simulink model "mars_rover_terrain"  (R2025a)
settings: Solver=daessc  StartTime=0.0  StopTime=130*10  FixedStep=1e-10  MaxStep=1e-1  RelTol=1e-3  AbsTol=1e-3  EnableMultiTasking=on
undefined symbols (not defined in the file): arm_q0, Control, eeConfig, L1, L2, L3, LS1, LS3, R1, R2, R3, Rover, rover_path, RS1, RS3, X, Y, Z
libraries: sm_lib x137, nesl_utility x109, fl_lib x85, sdl_lib x20, ee_lib x10, mars_rover_lib x8, simulink x4, slpidlib x3, batteryecm_lib x2, robotcorelib x1, robotalgslib x1
(part 7 of 10)

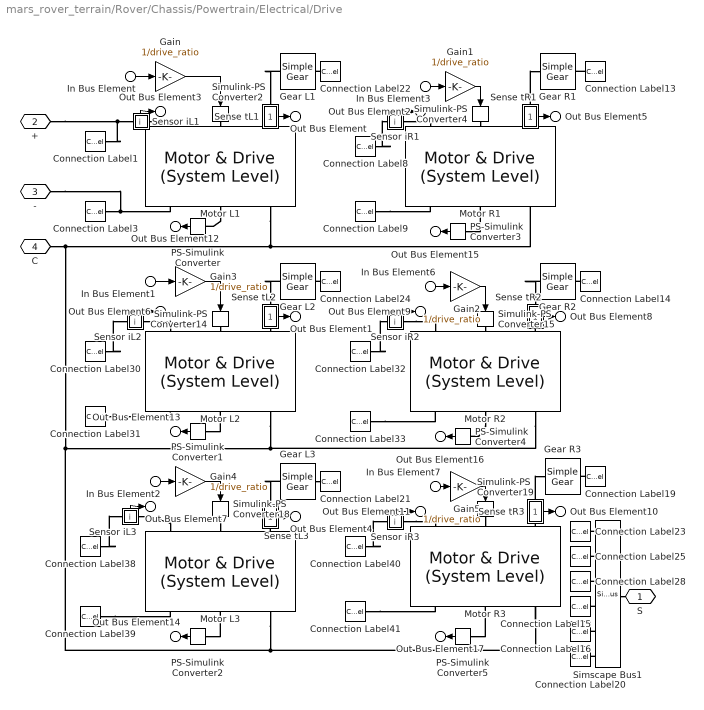
== system mars_rover_terrain/Rover/Chassis/Powertrain/Electrical/Drive ==
  In Bus Element : Inport  PortName=Trq  Element=trq.L1
  In Bus Element1 : Inport  PortName=Trq  Element=trq.L2
  In Bus Element2 : Inport  PortName=Trq  Element=trq.L3
  In Bus Element3 : Inport  PortName=Trq  Element=trq.R1
  In Bus Element6 : Inport  PortName=Trq  Element=trq.R2
  In Bus Element7 : Inport  PortName=Trq  Element=trq.R3
  Connection Label{1,8,30,32,38,40} (6 alike) : ConnectionLabel  Label=p
  Connection Label13 : ConnectionLabel  Label=R1
  Connection Label14 : ConnectionLabel  Label=R2
  Connection Label15 : ConnectionLabel  Label=R1
  Connection Label16 : ConnectionLabel  Label=R2
  Connection Label19 : ConnectionLabel  Label=R3
  Connection Label20 : ConnectionLabel  Label=R3
  Connection Label21 : ConnectionLabel  Label=L3
  Connection Label22 : ConnectionLabel  Label=L1
  Connection Label23 : ConnectionLabel  Label=L1
  Connection Label24 : ConnectionLabel  Label=L2
  Connection Label25 : ConnectionLabel  Label=L2
  Connection Label28 : ConnectionLabel  Label=L3
  Connection Label{3,9,31,33,39,41} (6 alike) : ConnectionLabel  Label=n
  Gain{,1..5} (6 alike) : Gain  Gain=1/drive_ratio
  Gear L2 : sdl_lib/Gears/Simple Gear  ratio=drive_ratio  rotation_direction=sdl.enum.shaftOutputDirection.same  friction_model=sdl.enum.gear_efficiencies_load.off  T_noload=0.1 N*m  T_nom=5 N*m  efficiency_nom=0.8  efficiency=drive_efficiency  temperature_TLU=[280, 300, 320] K  load_TLU=[1, 5, 10] N*m  efficiency_TLU=[.95, .9, .85]  efficiency_TLU2=[.85, .8, .75; .95, .9, .85; .85, .8, .7]  w_thr=0.01 rad/s  pwr_thr=0.001 W  enable_backlash=false  hardstop_model=simscape.enum.hardstop.smooth  backlash_distance=1e-3 mm  r_base=0.1 m  transition=1e-4 mm  backlash_stiffness=1e7 N/m  backlash_damping=1e6 N/(m/s)  coeff_rest=0  v_tol=0.001 m/s  f_tol=0 N  mu_visc=[0, 0] N*m/(rad/s)  thermal_mass=50 J/K  temperature_specify=off  temperature_priority=High  temperature=300 K  temperature_nominal_specify=off  temperature_nominal_value=1  temperature_nominal_unit=K  x_backlash_specify=off  x_backlash_priority=None  x_backlash=0 mm  x_backlash_nominal_specify=off  x_backlash_nominal_value=1  x_backlash_nominal_unit=mm  f_hardstop_specify=off  f_hardstop_priority=None  f_hardstop=0 N  f_hardstop_nominal_specify=off  f_hardstop_nominal_value=1  f_hardstop_nominal_unit=N  v_backlash_specify=off  v_backlash_priority=None  v_backlash=0 m/s  v_backlash_nominal_specify=off  v_backlash_nominal_value=1  v_backlash_nominal_unit=m/s
  Gear L3 : sdl_lib/Gears/Simple Gear  ratio=drive_ratio  rotation_direction=sdl.enum.shaftOutputDirection.same  friction_model=sdl.enum.gear_efficiencies_load.off  T_noload=0.1 N*m  T_nom=5 N*m  efficiency_nom=0.8  efficiency=drive_efficiency  temperature_TLU=[280, 300, 320] K  load_TLU=[1, 5, 10] N*m  efficiency_TLU=[.95, .9, .85]  efficiency_TLU2=[.85, .8, .75; .95, .9, .85; .85, .8, .7]  w_thr=0.01 rad/s  pwr_thr=0.001 W  enable_backlash=false  hardstop_model=simscape.enum.hardstop.smooth  backlash_distance=1e-3 mm  r_base=0.1 m  transition=1e-4 mm  backlash_stiffness=1e7 N/m  backlash_damping=1e6 N/(m/s)  coeff_rest=0  v_tol=0.001 m/s  f_tol=0 N  mu_visc=[0, 0] N*m/(rad/s)  thermal_mass=50 J/K  temperature_specify=off  temperature_priority=High  temperature=300 K  temperature_nominal_specify=off  temperature_nominal_value=1  temperature_nominal_unit=K  x_backlash_specify=off  x_backlash_priority=None  x_backlash=0 mm  x_backlash_nominal_specify=off  x_backlash_nominal_value=1  x_backlash_nominal_unit=mm  f_hardstop_specify=off  f_hardstop_priority=None  f_hardstop=0 N  f_hardstop_nominal_specify=off  f_hardstop_nominal_value=1  f_hardstop_nominal_unit=N  v_backlash_specify=off  v_backlash_priority=None  v_backlash=0 m/s  v_backlash_nominal_specify=off  v_backlash_nominal_value=1  v_backlash_nominal_unit=m/s
  Gear R1 : sdl_lib/Gears/Simple Gear  ratio=drive_ratio  rotation_direction=sdl.enum.shaftOutputDirection.same  friction_model=sdl.enum.gear_efficiencies_load.off  T_noload=0.1 N*m  T_nom=5 N*m  efficiency_nom=0.8  efficiency=drive_efficiency  temperature_TLU=[280, 300, 320] K  load_TLU=[1, 5, 10] N*m  efficiency_TLU=[.95, .9, .85]  efficiency_TLU2=[.85, .8, .75; .95, .9, .85; .85, .8, .7]  w_thr=0.01 rad/s  pwr_thr=0.001 W  enable_backlash=false  hardstop_model=simscape.enum.hardstop.smooth  backlash_distance=1e-3 mm  r_base=0.1 m  transition=1e-4 mm  backlash_stiffness=1e7 N/m  backlash_damping=1e6 N/(m/s)  coeff_rest=0  v_tol=0.001 m/s  f_tol=0 N  mu_visc=[0, 0] N*m/(rad/s)  thermal_mass=50 J/K  temperature_specify=off  temperature_priority=High  temperature=300 K  temperature_nominal_specify=off  temperature_nominal_value=1  temperature_nominal_unit=K  x_backlash_specify=off  x_backlash_priority=None  x_backlash=0 mm  x_backlash_nominal_specify=off  x_backlash_nominal_value=1  x_backlash_nominal_unit=mm  f_hardstop_specify=off  f_hardstop_priority=None  f_hardstop=0 N  f_hardstop_nominal_specify=off  f_hardstop_nominal_value=1  f_hardstop_nominal_unit=N  v_backlash_specify=off  v_backlash_priority=None  v_backlash=0 m/s  v_backlash_nominal_specify=off  v_backlash_nominal_value=1  v_backlash_nominal_unit=m/s
  Gear R2 : sdl_lib/Gears/Simple Gear  ratio=drive_ratio  rotation_direction=sdl.enum.shaftOutputDirection.same  friction_model=sdl.enum.gear_efficiencies_load.off  T_noload=0.1 N*m  T_nom=5 N*m  efficiency_nom=0.8  efficiency=drive_efficiency  temperature_TLU=[280, 300, 320] K  load_TLU=[1, 5, 10] N*m  efficiency_TLU=[.95, .9, .85]  efficiency_TLU2=[.85, .8, .75; .95, .9, .85; .85, .8, .7]  w_thr=0.01 rad/s  pwr_thr=0.001 W  enable_backlash=false  hardstop_model=simscape.enum.hardstop.smooth  backlash_distance=1e-3 mm  r_base=0.1 m  transition=1e-4 mm  backlash_stiffness=1e7 N/m  backlash_damping=1e6 N/(m/s)  coeff_rest=0  v_tol=0.001 m/s  f_tol=0 N  mu_visc=[0, 0] N*m/(rad/s)  thermal_mass=50 J/K  temperature_specify=off  temperature_priority=High  temperature=300 K  temperature_nominal_specify=off  temperature_nominal_value=1  temperature_nominal_unit=K  x_backlash_specify=off  x_backlash_priority=None  x_backlash=0 mm  x_backlash_nominal_specify=off  x_backlash_nominal_value=1  x_backlash_nominal_unit=mm  f_hardstop_specify=off  f_hardstop_priority=None  f_hardstop=0 N  f_hardstop_nominal_specify=off  f_hardstop_nominal_value=1  f_hardstop_nominal_unit=N  v_backlash_specify=off  v_backlash_priority=None  v_backlash=0 m/s  v_backlash_nominal_specify=off  v_backlash_nominal_value=1  v_backlash_nominal_unit=m/s
  Gear R3 : sdl_lib/Gears/Simple Gear  ratio=drive_ratio  rotation_direction=sdl.enum.shaftOutputDirection.same  friction_model=sdl.enum.gear_efficiencies_load.off  T_noload=0.1 N*m  T_nom=5 N*m  efficiency_nom=0.8  efficiency=drive_efficiency  temperature_TLU=[280, 300, 320] K  load_TLU=[1, 5, 10] N*m  efficiency_TLU=[.95, .9, .85]  efficiency_TLU2=[.85, .8, .75; .95, .9, .85; .85, .8, .7]  w_thr=0.01 rad/s  pwr_thr=0.001 W  enable_backlash=false  hardstop_model=simscape.enum.hardstop.smooth  backlash_distance=1e-3 mm  r_base=0.1 m  transition=1e-4 mm  backlash_stiffness=1e7 N/m  backlash_damping=1e6 N/(m/s)  coeff_rest=0  v_tol=0.001 m/s  f_tol=0 N  mu_visc=[0, 0] N*m/(rad/s)  thermal_mass=50 J/K  temperature_specify=off  temperature_priority=High  temperature=300 K  temperature_nominal_specify=off  temperature_nominal_value=1  temperature_nominal_unit=K  x_backlash_specify=off  x_backlash_priority=None  x_backlash=0 mm  x_backlash_nominal_specify=off  x_backlash_nominal_value=1  x_backlash_nominal_unit=mm  f_hardstop_specify=off  f_hardstop_priority=None  f_hardstop=0 N  f_hardstop_nominal_specify=off  f_hardstop_nominal_value=1  f_hardstop_nominal_unit=N  v_backlash_specify=off  v_backlash_priority=None  v_backlash=0 m/s  v_backlash_nominal_specify=off  v_backlash_nominal_value=1  v_backlash_nominal_unit=m/s
  Gear L1 : sdl_lib/Gears/Simple Gear  ratio=drive_ratio  rotation_direction=sdl.enum.shaftOutputDirection.same  friction_model=sdl.enum.gear_efficiencies_load.off  T_noload=0.1 N*m  T_nom=5 N*m  efficiency_nom=0.8  efficiency=drive_efficiency  temperature_TLU=[280, 300, 320] K  load_TLU=[1, 5, 10] N*m  efficiency_TLU=[.95, .9, .85]  efficiency_TLU2=[.85, .8, .75; .95, .9, .85; .85, .8, .7]  w_thr=0.01 rad/s  pwr_thr=0.001 W  enable_backlash=false  hardstop_model=simscape.enum.hardstop.smooth  backlash_distance=1e-3 mm  r_base=0.1 m  transition=1e-4 mm  backlash_stiffness=1e7 N/m  backlash_damping=1e6 N/(m/s)  coeff_rest=0  v_tol=0.001 m/s  f_tol=0 N  mu_visc=[0, 0] N*m/(rad/s)  thermal_mass=50 J/K  temperature_specify=off  temperature_priority=High  temperature=300 K  temperature_nominal_specify=off  temperature_nominal_value=1  temperature_nominal_unit=K  x_backlash_specify=off  x_backlash_priority=None  x_backlash=0 mm  x_backlash_nominal_specify=off  x_backlash_nominal_value=1  x_backlash_nominal_unit=mm  f_hardstop_specify=off  f_hardstop_priority=None  f_hardstop=0 N  f_hardstop_nominal_specify=off  f_hardstop_nominal_value=1  f_hardstop_nominal_unit=N  v_backlash_specify=off  v_backlash_priority=None  v_backlash=0 m/s  v_backlash_nominal_specify=off  v_backlash_nominal_value=1  v_backlash_nominal_unit=m/s
  Motor L1 : ee_lib/Electromechanical/Motor & Drive (System Level)  torque_speed_param=ee.enum.electromech.envelope.torque_power  overtorque_param=ee.enum.electromech.overtorque.no  T_t=[.09, .08, .07, 0] N*m  T_t_intermittent=[.36, .32, .28, 0] N*m  T_t_2D=[.09, .09, .09; .08, .08, .08; .07, .07, .07; 0, 0, 0] N*m  T_t_intermittent_2D=[.36, .36, .36; .32, .32, .32; .28, .28, .28; 0, 0, 0] N*m  w_t=[0, 3750, 7500, 8000] rpm  vdc_t=[6, 12, 24] V  torque_max=trq_max N*m  power_max=power_max W  torque_max_intermittent=0.4 N*m  power_max_intermittent=120 W  time_overtorque=30 s  time_recover=60 s  Tc=trq_tc s  EnableSwitch=simscape.enum.onoff.off  losses_param=1  eff=eff_overall  w_eff=eff_spd rpm  T_eff=eff_trq N*m  Piron=0 % not important in first iteration W  Pbase=0 % not important in first iteration W  w_eff_vec=[-8000, -4000, 0, 4000, 8000] rpm  T_eff_vec=[0, .03, .06, .09] N*m  v_eff_vec=[100, 250, 400] V  losses_mat=[1.49, 1.67, 2.21, 3.1; .42, .69, 1.14, 2.03; .06, .24, .78, 1.68; .42, .69, 1.14, 2.03; 1.49, 1.67, 2.21, 3.1] W  efficiency_mat=[95, 95, 95, 95; 95, 95, 95, 95; 95, 95, 95, 95; 95, 95, 95, 95; 95, 95, 95, 95]  losses_mat_3D=ones(5, 4, 3) W  efficiency_mat_3D=95 * ones(5, 4, 3)  Res=0 % not important in first iteration Ohm  J=0 kg*m^2  lam=rotor_d N*m/(rad/s)  speed0=0 rpm  faulted_specify=off  faulted_priority=None  faulted=0  faulted_nominal_specify=off  faulted_nominal_value=1  faulted_nominal_unit=1  isSwitchedOff_specify=off  isSwitchedOff_priority=None  isSwitchedOff=0  isSwitchedOff_nominal_specify=off  isSwitchedOff_nominal_value=1  isSwitchedOff_nominal_unit=1  torqueLimitContinuous_specify=off  torqueLimitContinuous_priority=None  torqueLimitContinuous=0 N*m  torqueLimitContinuous_nominal_specify=off  torqueLimitContinuous_nominal_value=1  torqueLimitContinuous_nominal_unit=N*m  alpha=3.93e-3 1/K  Tmeas=25 degC  Tmeas2=125 degC  losses_mat_T2=[1.49, 1.74, 2.49, 3.74; .42, .67, 1.42, 2.67; .06, .31, 1.06, 2.31; .42, .67, 1.42, 2.67; 1.49, 1.74, 2.49, 3.74] W  efficiency_mat_T2=[95, 95, 95, 95; 95, 95, 95, 95; 95, 95, 95, 95; 95, 95, 95, 95; 95, 95, 95, 95]  losses_mat_3D_T2=ones(5, 4, 3) W  efficiency_mat_3D_T2=95 * ones(5, 4, 3)  thermal_mass=100 J/K  initial_temperature=25 degC
  Motor L2 : ee_lib/Electromechanical/Motor & Drive (System Level)  torque_speed_param=ee.enum.electromech.envelope.torque_power  overtorque_param=ee.enum.electromech.overtorque.no  T_t=[.09, .08, .07, 0] N*m  T_t_intermittent=[.36, .32, .28, 0] N*m  T_t_2D=[.09, .09, .09; .08, .08, .08; .07, .07, .07; 0, 0, 0] N*m  T_t_intermittent_2D=[.36, .36, .36; .32, .32, .32; .28, .28, .28; 0, 0, 0] N*m  w_t=[0, 3750, 7500, 8000] rpm  vdc_t=[6, 12, 24] V  torque_max=trq_max N*m  power_max=power_max W  torque_max_intermittent=0.4 N*m  power_max_intermittent=120 W  time_overtorque=30 s  time_recover=60 s  Tc=trq_tc s  EnableSwitch=simscape.enum.onoff.off  losses_param=1  eff=eff_overall  w_eff=eff_spd rpm  T_eff=eff_trq N*m  Piron=0 % not important in first iteration W  Pbase=0 % not important in first iteration W  w_eff_vec=[-8000, -4000, 0, 4000, 8000] rpm  T_eff_vec=[0, .03, .06, .09] N*m  v_eff_vec=[100, 250, 400] V  losses_mat=[1.49, 1.67, 2.21, 3.1; .42, .69, 1.14, 2.03; .06, .24, .78, 1.68; .42, .69, 1.14, 2.03; 1.49, 1.67, 2.21, 3.1] W  efficiency_mat=[95, 95, 95, 95; 95, 95, 95, 95; 95, 95, 95, 95; 95, 95, 95, 95; 95, 95, 95, 95]  losses_mat_3D=ones(5, 4, 3) W  efficiency_mat_3D=95 * ones(5, 4, 3)  Res=0 % not important in first iteration Ohm  J=0 kg*m^2  lam=rotor_d N*m/(rad/s)  speed0=0 rpm  faulted_specify=off  faulted_priority=None  faulted=0  faulted_nominal_specify=off  faulted_nominal_value=1  faulted_nominal_unit=1  isSwitchedOff_specify=off  isSwitchedOff_priority=None  isSwitchedOff=0  isSwitchedOff_nominal_specify=off  isSwitchedOff_nominal_value=1  isSwitchedOff_nominal_unit=1  torqueLimitContinuous_specify=off  torqueLimitContinuous_priority=None  torqueLimitContinuous=0 N*m  torqueLimitContinuous_nominal_specify=off  torqueLimitContinuous_nominal_value=1  torqueLimitContinuous_nominal_unit=N*m  alpha=3.93e-3 1/K  Tmeas=25 degC  Tmeas2=125 degC  losses_mat_T2=[1.49, 1.74, 2.49, 3.74; .42, .67, 1.42, 2.67; .06, .31, 1.06, 2.31; .42, .67, 1.42, 2.67; 1.49, 1.74, 2.49, 3.74] W  efficiency_mat_T2=[95, 95, 95, 95; 95, 95, 95, 95; 95, 95, 95, 95; 95, 95, 95, 95; 95, 95, 95, 95]  losses_mat_3D_T2=ones(5, 4, 3) W  efficiency_mat_3D_T2=95 * ones(5, 4, 3)  thermal_mass=100 J/K  initial_temperature=25 degC
  Motor L3 : ee_lib/Electromechanical/Motor & Drive (System Level)  torque_speed_param=ee.enum.electromech.envelope.torque_power  overtorque_param=ee.enum.electromech.overtorque.no  T_t=[.09, .08, .07, 0] N*m  T_t_intermittent=[.36, .32, .28, 0] N*m  T_t_2D=[.09, .09, .09; .08, .08, .08; .07, .07, .07; 0, 0, 0] N*m  T_t_intermittent_2D=[.36, .36, .36; .32, .32, .32; .28, .28, .28; 0, 0, 0] N*m  w_t=[0, 3750, 7500, 8000] rpm  vdc_t=[6, 12, 24] V  torque_max=trq_max N*m  power_max=power_max W  torque_max_intermittent=0.4 N*m  power_max_intermittent=120 W  time_overtorque=30 s  time_recover=60 s  Tc=trq_tc s  EnableSwitch=simscape.enum.onoff.off  losses_param=1  eff=eff_overall  w_eff=eff_spd rpm  T_eff=eff_trq N*m  Piron=0 % not important in first iteration W  Pbase=0 % not important in first iteration W  w_eff_vec=[-8000, -4000, 0, 4000, 8000] rpm  T_eff_vec=[0, .03, .06, .09] N*m  v_eff_vec=[100, 250, 400] V  losses_mat=[1.49, 1.67, 2.21, 3.1; .42, .69, 1.14, 2.03; .06, .24, .78, 1.68; .42, .69, 1.14, 2.03; 1.49, 1.67, 2.21, 3.1] W  efficiency_mat=[95, 95, 95, 95; 95, 95, 95, 95; 95, 95, 95, 95; 95, 95, 95, 95; 95, 95, 95, 95]  losses_mat_3D=ones(5, 4, 3) W  efficiency_mat_3D=95 * ones(5, 4, 3)  Res=0 % not important in first iteration Ohm  J=0 kg*m^2  lam=rotor_d N*m/(rad/s)  speed0=0 rpm  faulted_specify=off  faulted_priority=None  faulted=0  faulted_nominal_specify=off  faulted_nominal_value=1  faulted_nominal_unit=1  isSwitchedOff_specify=off  isSwitchedOff_priority=None  isSwitchedOff=0  isSwitchedOff_nominal_specify=off  isSwitchedOff_nominal_value=1  isSwitchedOff_nominal_unit=1  torqueLimitContinuous_specify=off  torqueLimitContinuous_priority=None  torqueLimitContinuous=0 N*m  torqueLimitContinuous_nominal_specify=off  torqueLimitContinuous_nominal_value=1  torqueLimitContinuous_nominal_unit=N*m  alpha=3.93e-3 1/K  Tmeas=25 degC  Tmeas2=125 degC  losses_mat_T2=[1.49, 1.74, 2.49, 3.74; .42, .67, 1.42, 2.67; .06, .31, 1.06, 2.31; .42, .67, 1.42, 2.67; 1.49, 1.74, 2.49, 3.74] W  efficiency_mat_T2=[95, 95, 95, 95; 95, 95, 95, 95; 95, 95, 95, 95; 95, 95, 95, 95; 95, 95, 95, 95]  losses_mat_3D_T2=ones(5, 4, 3) W  efficiency_mat_3D_T2=95 * ones(5, 4, 3)  thermal_mass=100 J/K  initial_temperature=25 degC
  Motor R1 : ee_lib/Electromechanical/Motor & Drive (System Level)  torque_speed_param=ee.enum.electromech.envelope.torque_power  overtorque_param=ee.enum.electromech.overtorque.no  T_t=[.09, .08, .07, 0] N*m  T_t_intermittent=[.36, .32, .28, 0] N*m  T_t_2D=[.09, .09, .09; .08, .08, .08; .07, .07, .07; 0, 0, 0] N*m  T_t_intermittent_2D=[.36, .36, .36; .32, .32, .32; .28, .28, .28; 0, 0, 0] N*m  w_t=[0, 3750, 7500, 8000] rpm  vdc_t=[6, 12, 24] V  torque_max=trq_max N*m  power_max=power_max W  torque_max_intermittent=0.4 N*m  power_max_intermittent=120 W  time_overtorque=30 s  time_recover=60 s  Tc=trq_tc s  EnableSwitch=simscape.enum.onoff.off  losses_param=1  eff=eff_overall  w_eff=eff_spd rpm  T_eff=eff_trq N*m  Piron=0 % not important in first iteration W  Pbase=0 % not important in first iteration W  w_eff_vec=[-8000, -4000, 0, 4000, 8000] rpm  T_eff_vec=[0, .03, .06, .09] N*m  v_eff_vec=[100, 250, 400] V  losses_mat=[1.49, 1.67, 2.21, 3.1; .42, .69, 1.14, 2.03; .06, .24, .78, 1.68; .42, .69, 1.14, 2.03; 1.49, 1.67, 2.21, 3.1] W  efficiency_mat=[95, 95, 95, 95; 95, 95, 95, 95; 95, 95, 95, 95; 95, 95, 95, 95; 95, 95, 95, 95]  losses_mat_3D=ones(5, 4, 3) W  efficiency_mat_3D=95 * ones(5, 4, 3)  Res=0 % not important in first iteration Ohm  J=0 kg*m^2  lam=rotor_d N*m/(rad/s)  speed0=0 rpm  faulted_specify=off  faulted_priority=None  faulted=0  faulted_nominal_specify=off  faulted_nominal_value=1  faulted_nominal_unit=1  isSwitchedOff_specify=off  isSwitchedOff_priority=None  isSwitchedOff=0  isSwitchedOff_nominal_specify=off  isSwitchedOff_nominal_value=1  isSwitchedOff_nominal_unit=1  torqueLimitContinuous_specify=off  torqueLimitContinuous_priority=None  torqueLimitContinuous=0 N*m  torqueLimitContinuous_nominal_specify=off  torqueLimitContinuous_nominal_value=1  torqueLimitContinuous_nominal_unit=N*m  alpha=3.93e-3 1/K  Tmeas=25 degC  Tmeas2=125 degC  losses_mat_T2=[1.49, 1.74, 2.49, 3.74; .42, .67, 1.42, 2.67; .06, .31, 1.06, 2.31; .42, .67, 1.42, 2.67; 1.49, 1.74, 2.49, 3.74] W  efficiency_mat_T2=[95, 95, 95, 95; 95, 95, 95, 95; 95, 95, 95, 95; 95, 95, 95, 95; 95, 95, 95, 95]  losses_mat_3D_T2=ones(5, 4, 3) W  efficiency_mat_3D_T2=95 * ones(5, 4, 3)  thermal_mass=100 J/K  initial_temperature=25 degC
  Motor R2 : ee_lib/Electromechanical/Motor & Drive (System Level)  torque_speed_param=ee.enum.electromech.envelope.torque_power  overtorque_param=ee.enum.electromech.overtorque.no  T_t=[.09, .08, .07, 0] N*m  T_t_intermittent=[.36, .32, .28, 0] N*m  T_t_2D=[.09, .09, .09; .08, .08, .08; .07, .07, .07; 0, 0, 0] N*m  T_t_intermittent_2D=[.36, .36, .36; .32, .32, .32; .28, .28, .28; 0, 0, 0] N*m  w_t=[0, 3750, 7500, 8000] rpm  vdc_t=[6, 12, 24] V  torque_max=trq_max N*m  power_max=power_max W  torque_max_intermittent=0.4 N*m  power_max_intermittent=120 W  time_overtorque=30 s  time_recover=60 s  Tc=trq_tc s  EnableSwitch=simscape.enum.onoff.off  losses_param=1  eff=eff_overall  w_eff=eff_spd rpm  T_eff=eff_trq N*m  Piron=0 % not important in first iteration W  Pbase=0 % not important in first iteration W  w_eff_vec=[-8000, -4000, 0, 4000, 8000] rpm  T_eff_vec=[0, .03, .06, .09] N*m  v_eff_vec=[100, 250, 400] V  losses_mat=[1.49, 1.67, 2.21, 3.1; .42, .69, 1.14, 2.03; .06, .24, .78, 1.68; .42, .69, 1.14, 2.03; 1.49, 1.67, 2.21, 3.1] W  efficiency_mat=[95, 95, 95, 95; 95, 95, 95, 95; 95, 95, 95, 95; 95, 95, 95, 95; 95, 95, 95, 95]  losses_mat_3D=ones(5, 4, 3) W  efficiency_mat_3D=95 * ones(5, 4, 3)  Res=0 % not important in first iteration Ohm  J=0 kg*m^2  lam=rotor_d N*m/(rad/s)  speed0=0 rpm  faulted_specify=off  faulted_priority=None  faulted=0  faulted_nominal_specify=off  faulted_nominal_value=1  faulted_nominal_unit=1  isSwitchedOff_specify=off  isSwitchedOff_priority=None  isSwitchedOff=0  isSwitchedOff_nominal_specify=off  isSwitchedOff_nominal_value=1  isSwitchedOff_nominal_unit=1  torqueLimitContinuous_specify=off  torqueLimitContinuous_priority=None  torqueLimitContinuous=0 N*m  torqueLimitContinuous_nominal_specify=off  torqueLimitContinuous_nominal_value=1  torqueLimitContinuous_nominal_unit=N*m  alpha=3.93e-3 1/K  Tmeas=25 degC  Tmeas2=125 degC  losses_mat_T2=[1.49, 1.74, 2.49, 3.74; .42, .67, 1.42, 2.67; .06, .31, 1.06, 2.31; .42, .67, 1.42, 2.67; 1.49, 1.74, 2.49, 3.74] W  efficiency_mat_T2=[95, 95, 95, 95; 95, 95, 95, 95; 95, 95, 95, 95; 95, 95, 95, 95; 95, 95, 95, 95]  losses_mat_3D_T2=ones(5, 4, 3) W  efficiency_mat_3D_T2=95 * ones(5, 4, 3)  thermal_mass=100 J/K  initial_temperature=25 degC
  Motor R3 : ee_lib/Electromechanical/Motor & Drive (System Level)  torque_speed_param=ee.enum.electromech.envelope.torque_power  overtorque_param=ee.enum.electromech.overtorque.no  T_t=[.09, .08, .07, 0] N*m  T_t_intermittent=[.36, .32, .28, 0] N*m  T_t_2D=[.09, .09, .09; .08, .08, .08; .07, .07, .07; 0, 0, 0] N*m  T_t_intermittent_2D=[.36, .36, .36; .32, .32, .32; .28, .28, .28; 0, 0, 0] N*m  w_t=[0, 3750, 7500, 8000] rpm  vdc_t=[6, 12, 24] V  torque_max=trq_max N*m  power_max=power_max W  torque_max_intermittent=0.4 N*m  power_max_intermittent=120 W  time_overtorque=30 s  time_recover=60 s  Tc=trq_tc s  EnableSwitch=simscape.enum.onoff.off  losses_param=1  eff=eff_overall  w_eff=eff_spd rpm  T_eff=eff_trq N*m  Piron=0 % not important in first iteration W  Pbase=0 % not important in first iteration W  w_eff_vec=[-8000, -4000, 0, 4000, 8000] rpm  T_eff_vec=[0, .03, .06, .09] N*m  v_eff_vec=[100, 250, 400] V  losses_mat=[1.49, 1.67, 2.21, 3.1; .42, .69, 1.14, 2.03; .06, .24, .78, 1.68; .42, .69, 1.14, 2.03; 1.49, 1.67, 2.21, 3.1] W  efficiency_mat=[95, 95, 95, 95; 95, 95, 95, 95; 95, 95, 95, 95; 95, 95, 95, 95; 95, 95, 95, 95]  losses_mat_3D=ones(5, 4, 3) W  efficiency_mat_3D=95 * ones(5, 4, 3)  Res=0 % not important in first iteration Ohm  J=0 kg*m^2  lam=rotor_d N*m/(rad/s)  speed0=0 rpm  faulted_specify=off  faulted_priority=None  faulted=0  faulted_nominal_specify=off  faulted_nominal_value=1  faulted_nominal_unit=1  isSwitchedOff_specify=off  isSwitchedOff_priority=None  isSwitchedOff=0  isSwitchedOff_nominal_specify=off  isSwitchedOff_nominal_value=1  isSwitchedOff_nominal_unit=1  torqueLimitContinuous_specify=off  torqueLimitContinuous_priority=None  torqueLimitContinuous=0 N*m  torqueLimitContinuous_nominal_specify=off  torqueLimitContinuous_nominal_value=1  torqueLimitContinuous_nominal_unit=N*m  alpha=3.93e-3 1/K  Tmeas=25 degC  Tmeas2=125 degC  losses_mat_T2=[1.49, 1.74, 2.49, 3.74; .42, .67, 1.42, 2.67; .06, .31, 1.06, 2.31; .42, .67, 1.42, 2.67; 1.49, 1.74, 2.49, 3.74] W  efficiency_mat_T2=[95, 95, 95, 95; 95, 95, 95, 95; 95, 95, 95, 95; 95, 95, 95, 95; 95, 95, 95, 95]  losses_mat_3D_T2=ones(5, 4, 3) W  efficiency_mat_3D_T2=95 * ones(5, 4, 3)  thermal_mass=100 J/K  initial_temperature=25 degC
  PS-Simulink Converter{,1..5} (6 alike) : nesl_utility/PS-Simulink Converter  PhysicalDomain=network_engine_domain  SubClassName=ps_output  LeftPortType=input  RightPortType=output  PseudoPeriodic=off  Frequencies=[]  VectorFormat=1-D array  Unit=inherit  AffineConversion=off
  Sense tL1 : Subsystem
      settings: PortSchema="{\"entries\":[{\"content\":{\"sides\":[{\"content\":{\"connectorIds\":[\"LConn1\"]},\"type\":\"ConnectorPlacement.EquallySpacedRectSide\",\"uuid\":\"592cc1a1-656f-47ce-ad3a-4b4dc1070b5c\"},{\"content\":{\"connectorIds\":[\"RConn1\"],\"side\":\"RIGHT\"},\"type\":\"ConnectorPlacement.EquallySpacedRectSide\",\"uuid\":\"9bca39c3-eeb4-4456-9b97-61ec2f027d42\"},{\"content\":{\"connectorIds\":[\"Out1\"],\"side\":\"TOP\"},\"type\":\"ConnectorPlacement.EquallySpacedRectSide\",\"uuid\":\"1e04bf27-fb0c-4be4-96d5-7a7c6152a7df\"}]},\"type\":\"ConnectorPlacement.EquallySpacedConnector\",\"uuid\":\"70eba8cc-e966-48e4-a1ce-5ccb9693dc60\"}],\"packageUris\":[\"http://schema.mathworks.com/mf0/Connector/R2020b\"],\"version\":\"1.0\"}"
      mask Display: disp('t')
  Sense tL2 : Subsystem
      settings: PortSchema="{\"entries\":[{\"content\":{\"sides\":[{\"content\":{\"connectorIds\":[\"LConn1\"]},\"type\":\"ConnectorPlacement.EquallySpacedRectSide\",\"uuid\":\"592cc1a1-656f-47ce-ad3a-4b4dc1070b5c\"},{\"content\":{\"connectorIds\":[\"RConn1\"],\"side\":\"RIGHT\"},\"type\":\"ConnectorPlacement.EquallySpacedRectSide\",\"uuid\":\"9bca39c3-eeb4-4456-9b97-61ec2f027d42\"},{\"content\":{\"connectorIds\":[\"Out1\"],\"side\":\"TOP\"},\"type\":\"ConnectorPlacement.EquallySpacedRectSide\",\"uuid\":\"1e04bf27-fb0c-4be4-96d5-7a7c6152a7df\"}]},\"type\":\"ConnectorPlacement.EquallySpacedConnector\",\"uuid\":\"70eba8cc-e966-48e4-a1ce-5ccb9693dc60\"}],\"packageUris\":[\"http://schema.mathworks.com/mf0/Connector/R2020b\"],\"version\":\"1.0\"}"
      mask Display: disp('t')
  Sense tL3 : Subsystem
      settings: PortSchema="{\"entries\":[{\"content\":{\"sides\":[{\"content\":{\"connectorIds\":[\"LConn1\"]},\"type\":\"ConnectorPlacement.EquallySpacedRectSide\",\"uuid\":\"592cc1a1-656f-47ce-ad3a-4b4dc1070b5c\"},{\"content\":{\"connectorIds\":[\"RConn1\"],\"side\":\"RIGHT\"},\"type\":\"ConnectorPlacement.EquallySpacedRectSide\",\"uuid\":\"9bca39c3-eeb4-4456-9b97-61ec2f027d42\"},{\"content\":{\"connectorIds\":[\"Out1\"],\"side\":\"TOP\"},\"type\":\"ConnectorPlacement.EquallySpacedRectSide\",\"uuid\":\"1e04bf27-fb0c-4be4-96d5-7a7c6152a7df\"},{\"content\":{\"connectorIds\":[],\"side\":\"BOTTOM\"},\"type\":\"ConnectorPlacement.EquallySpacedRectSide\",\"uuid\":\"710085da-f7c8-4ce8-b21c-6bd8281c2790\"}]},\"type\":\"ConnectorPlacement.EquallySpacedConnector\",\"uuid\":\"70eba8cc-e966-48e4-a1ce-5ccb9693dc60\"}],\"packageUris\":[\"http://schema.mathworks.com/mf0/Connector/R2020b\"],\"version\":\"1.0\"}"
      mask Display: disp('t')
  Sense tR1 : Subsystem
      settings: PortSchema="{\"entries\":[{\"content\":{\"sides\":[{\"content\":{\"connectorIds\":[\"LConn1\"]},\"type\":\"ConnectorPlacement.EquallySpacedRectSide\",\"uuid\":\"592cc1a1-656f-47ce-ad3a-4b4dc1070b5c\"},{\"content\":{\"connectorIds\":[\"RConn1\"],\"side\":\"RIGHT\"},\"type\":\"ConnectorPlacement.EquallySpacedRectSide\",\"uuid\":\"9bca39c3-eeb4-4456-9b97-61ec2f027d42\"},{\"content\":{\"connectorIds\":[\"Out1\"],\"side\":\"TOP\"},\"type\":\"ConnectorPlacement.EquallySpacedRectSide\",\"uuid\":\"1e04bf27-fb0c-4be4-96d5-7a7c6152a7df\"}]},\"type\":\"ConnectorPlacement.EquallySpacedConnector\",\"uuid\":\"70eba8cc-e966-48e4-a1ce-5ccb9693dc60\"}],\"packageUris\":[\"http://schema.mathworks.com/mf0/Connector/R2020b\"],\"version\":\"1.0\"}"
      mask Display: disp('t')
  Sense tR2 : Subsystem
      settings: PortSchema="{\"entries\":[{\"content\":{\"sides\":[{\"content\":{\"connectorIds\":[\"LConn1\"]},\"type\":\"ConnectorPlacement.EquallySpacedRectSide\",\"uuid\":\"592cc1a1-656f-47ce-ad3a-4b4dc1070b5c\"},{\"content\":{\"connectorIds\":[\"RConn1\"],\"side\":\"RIGHT\"},\"type\":\"ConnectorPlacement.EquallySpacedRectSide\",\"uuid\":\"9bca39c3-eeb4-4456-9b97-61ec2f027d42\"},{\"content\":{\"connectorIds\":[\"Out1\"],\"side\":\"TOP\"},\"type\":\"ConnectorPlacement.EquallySpacedRectSide\",\"uuid\":\"1e04bf27-fb0c-4be4-96d5-7a7c6152a7df\"}]},\"type\":\"ConnectorPlacement.EquallySpacedConnector\",\"uuid\":\"70eba8cc-e966-48e4-a1ce-5ccb9693dc60\"}],\"packageUris\":[\"http://schema.mathworks.com/mf0/Connector/R2020b\"],\"version\":\"1.0\"}"
      mask Display: disp('t')
  Sense tR3 : Subsystem
      settings: PortSchema="{\"entries\":[{\"content\":{\"sides\":[{\"content\":{\"connectorIds\":[\"LConn1\"]},\"type\":\"ConnectorPlacement.EquallySpacedRectSide\",\"uuid\":\"592cc1a1-656f-47ce-ad3a-4b4dc1070b5c\"},{\"content\":{\"connectorIds\":[\"RConn1\"],\"side\":\"RIGHT\"},\"type\":\"ConnectorPlacement.EquallySpacedRectSide\",\"uuid\":\"9bca39c3-eeb4-4456-9b97-61ec2f027d42\"},{\"content\":{\"connectorIds\":[\"Out1\"],\"side\":\"TOP\"},\"type\":\"ConnectorPlacement.EquallySpacedRectSide\",\"uuid\":\"1e04bf27-fb0c-4be4-96d5-7a7c6152a7df\"}]},\"type\":\"ConnectorPlacement.EquallySpacedConnector\",\"uuid\":\"70eba8cc-e966-48e4-a1ce-5ccb9693dc60\"}],\"packageUris\":[\"http://schema.mathworks.com/mf0/Connector/R2020b\"],\"version\":\"1.0\"}"
      mask Display: disp('t')
  Sensor iL1 : Subsystem
      settings: PortSchema="{\"entries\":[{\"content\":{\"sides\":[{\"content\":{\"connectorIds\":[\"LConn1\"]},\"type\":\"ConnectorPlacement.EquallySpacedRectSide\",\"uuid\":\"592cc1a1-656f-47ce-ad3a-4b4dc1070b5c\"},{\"content\":{\"connectorIds\":[\"RConn1\"],\"side\":\"RIGHT\"},\"type\":\"ConnectorPlacement.EquallySpacedRectSide\",\"uuid\":\"9bca39c3-eeb4-4456-9b97-61ec2f027d42\"},{\"content\":{\"connectorIds\":[\"Out1\"],\"side\":\"TOP\"},\"type\":\"ConnectorPlacement.EquallySpacedRectSide\",\"uuid\":\"1e04bf27-fb0c-4be4-96d5-7a7c6152a7df\"}]},\"type\":\"ConnectorPlacement.EquallySpacedConnector\",\"uuid\":\"70eba8cc-e966-48e4-a1ce-5ccb9693dc60\"}],\"packageUris\":[\"http://schema.mathworks.com/mf0/Connector/R2020b\"],\"version\":\"1.0\"}"
      mask Display: disp('i');
  Sensor iL2 : Subsystem
      settings: PortSchema="{\"entries\":[{\"content\":{\"sides\":[{\"content\":{\"connectorIds\":[\"LConn1\"]},\"type\":\"ConnectorPlacement.EquallySpacedRectSide\",\"uuid\":\"592cc1a1-656f-47ce-ad3a-4b4dc1070b5c\"},{\"content\":{\"connectorIds\":[\"RConn1\"],\"side\":\"RIGHT\"},\"type\":\"ConnectorPlacement.EquallySpacedRectSide\",\"uuid\":\"9bca39c3-eeb4-4456-9b97-61ec2f027d42\"},{\"content\":{\"connectorIds\":[\"Out1\"],\"side\":\"TOP\"},\"type\":\"ConnectorPlacement.EquallySpacedRectSide\",\"uuid\":\"1e04bf27-fb0c-4be4-96d5-7a7c6152a7df\"}]},\"type\":\"ConnectorPlacement.EquallySpacedConnector\",\"uuid\":\"70eba8cc-e966-48e4-a1ce-5ccb9693dc60\"}],\"packageUris\":[\"http://schema.mathworks.com/mf0/Connector/R2020b\"],\"version\":\"1.0\"}"
      mask Display: disp('i');
  Sensor iL3 : Subsystem
      settings: PortSchema="{\"entries\":[{\"content\":{\"sides\":[{\"content\":{\"connectorIds\":[\"LConn1\"]},\"type\":\"ConnectorPlacement.EquallySpacedRectSide\",\"uuid\":\"592cc1a1-656f-47ce-ad3a-4b4dc1070b5c\"},{\"content\":{\"connectorIds\":[\"RConn1\"],\"side\":\"RIGHT\"},\"type\":\"ConnectorPlacement.EquallySpacedRectSide\",\"uuid\":\"9bca39c3-eeb4-4456-9b97-61ec2f027d42\"},{\"content\":{\"connectorIds\":[\"Out1\"],\"side\":\"TOP\"},\"type\":\"ConnectorPlacement.EquallySpacedRectSide\",\"uuid\":\"1e04bf27-fb0c-4be4-96d5-7a7c6152a7df\"}]},\"type\":\"ConnectorPlacement.EquallySpacedConnector\",\"uuid\":\"70eba8cc-e966-48e4-a1ce-5ccb9693dc60\"}],\"packageUris\":[\"http://schema.mathworks.com/mf0/Connector/R2020b\"],\"version\":\"1.0\"}"
      mask Display: disp('i');
  Sensor iR1 : Subsystem
      settings: PortSchema="{\"entries\":[{\"content\":{\"sides\":[{\"content\":{\"connectorIds\":[\"LConn1\"]},\"type\":\"ConnectorPlacement.EquallySpacedRectSide\",\"uuid\":\"592cc1a1-656f-47ce-ad3a-4b4dc1070b5c\"},{\"content\":{\"connectorIds\":[\"RConn1\"],\"side\":\"RIGHT\"},\"type\":\"ConnectorPlacement.EquallySpacedRectSide\",\"uuid\":\"9bca39c3-eeb4-4456-9b97-61ec2f027d42\"},{\"content\":{\"connectorIds\":[\"Out1\"],\"side\":\"TOP\"},\"type\":\"ConnectorPlacement.EquallySpacedRectSide\",\"uuid\":\"1e04bf27-fb0c-4be4-96d5-7a7c6152a7df\"}]},\"type\":\"ConnectorPlacement.EquallySpacedConnector\",\"uuid\":\"70eba8cc-e966-48e4-a1ce-5ccb9693dc60\"}],\"packageUris\":[\"http://schema.mathworks.com/mf0/Connector/R2020b\"],\"version\":\"1.0\"}"
      mask Display: disp('i');
  Sensor iR2 : Subsystem
      settings: PortSchema="{\"entries\":[{\"content\":{\"sides\":[{\"content\":{\"connectorIds\":[\"LConn1\"]},\"type\":\"ConnectorPlacement.EquallySpacedRectSide\",\"uuid\":\"592cc1a1-656f-47ce-ad3a-4b4dc1070b5c\"},{\"content\":{\"connectorIds\":[\"RConn1\"],\"side\":\"RIGHT\"},\"type\":\"ConnectorPlacement.EquallySpacedRectSide\",\"uuid\":\"9bca39c3-eeb4-4456-9b97-61ec2f027d42\"},{\"content\":{\"connectorIds\":[\"Out1\"],\"side\":\"TOP\"},\"type\":\"ConnectorPlacement.EquallySpacedRectSide\",\"uuid\":\"1e04bf27-fb0c-4be4-96d5-7a7c6152a7df\"}]},\"type\":\"ConnectorPlacement.EquallySpacedConnector\",\"uuid\":\"70eba8cc-e966-48e4-a1ce-5ccb9693dc60\"}],\"packageUris\":[\"http://schema.mathworks.com/mf0/Connector/R2020b\"],\"version\":\"1.0\"}"
      mask Display: disp('i');
  Sensor iR3 : Subsystem
      settings: PortSchema="{\"entries\":[{\"content\":{\"sides\":[{\"content\":{\"connectorIds\":[\"LConn1\"]},\"type\":\"ConnectorPlacement.EquallySpacedRectSide\",\"uuid\":\"592cc1a1-656f-47ce-ad3a-4b4dc1070b5c\"},{\"content\":{\"connectorIds\":[\"RConn1\"],\"side\":\"RIGHT\"},\"type\":\"ConnectorPlacement.EquallySpacedRectSide\",\"uuid\":\"9bca39c3-eeb4-4456-9b97-61ec2f027d42\"},{\"content\":{\"connectorIds\":[\"Out1\"],\"side\":\"TOP\"},\"type\":\"ConnectorPlacement.EquallySpacedRectSide\",\"uuid\":\"1e04bf27-fb0c-4be4-96d5-7a7c6152a7df\"}]},\"type\":\"ConnectorPlacement.EquallySpacedConnector\",\"uuid\":\"70eba8cc-e966-48e4-a1ce-5ccb9693dc60\"}],\"packageUris\":[\"http://schema.mathworks.com/mf0/Connector/R2020b\"],\"version\":\"1.0\"}"
      mask Display: disp('i');
  Simscape Bus1 : SimscapeBus  HierarchyStrings=L1;L2;L3;R1;R2;R3
  Simulink-PS Converter{2,4,14..15,18..19} (6 alike) : nesl_utility/Simulink-PS Converter  PhysicalDomain=network_engine_domain  SubClassName=ps_input  LeftPortType=input  RightPortType=output  PseudoPeriodic=off  Frequencies=[]  NoiseDistribution=none  NoiseParameters=[]  Unit=N*m  AffineConversion=off  FilteringAndDerivatives=provide  SimscapeFilterOrder=1  InputFilterTimeConstant=0.001  UdotUserProvided=0
  S : PMIOPort  Side=Right
  + : PMIOPort  Port=2  Side=Left
  - : PMIOPort  Port=3  Side=Left
  C : PMIOPort  Port=4  Side=Right
  Out Bus Element : Outport  PortName=m  Element=trq.L1
  Out Bus Element1 : Outport  PortName=m  Element=trq.L2
  Out Bus Element4 : Outport  PortName=m  Element=trq.L3
  Out Bus Element5 : Outport  PortName=m  Element=trq.R1
  Out Bus Element8 : Outport  PortName=m  Element=trq.R2
  Out Bus Element10 : Outport  PortName=m  Element=trq.R3
  Out Bus Element3 : Outport  PortName=m  Element=i.L1
  Out Bus Element6 : Outport  PortName=m  Element=i.L2
  Out Bus Element7 : Outport  PortName=m  Element=i.L3
  Out Bus Element2 : Outport  PortName=m  Element=i.R1
  Out Bus Element9 : Outport  PortName=m  Element=i.R2
  Out Bus Element11 : Outport  PortName=m  Element=i.R3
  Out Bus Element12 : Outport  PortName=m  Element=w.L1
  Out Bus Element13 : Outport  PortName=m  Element=w.L2
  Out Bus Element14 : Outport  PortName=m  Element=w.L3
  Out Bus Element15 : Outport  PortName=m  Element=w.R1
  Out Bus Element16 : Outport  PortName=m  Element=w.R2
  Out Bus Element17 : Outport  PortName=m  Element=w.R3
  wires:
  Sensor iR2/1(i) -> Out Bus Element9/1
  Sensor iL1/1(i) -> Out Bus Element3/1
  Sensor iL3/1(i) -> Out Bus Element7/1
  Sensor iL2/1(i) -> Out Bus Element6/1
  Sensor iR1/1(i) -> Out Bus Element2/1
  In Bus Element/1 -> Gain/1
  In Bus Element1/1 -> Gain3/1
  In Bus Element2/1 -> Gain4/1
  In Bus Element3/1 -> Gain1/1
  In Bus Element6/1 -> Gain2/1
  In Bus Element7/1 -> Gain5/1
  Sensor iR3/1(i) -> Out Bus Element11/1
  Gain/1 -> Simulink-PS Converter2/1
  Gain1/1 -> Simulink-PS Converter4/1
  Gain2/1 -> Simulink-PS Converter15/1
  Gain3/1 -> Simulink-PS Converter14/1
  Gain4/1 -> Simulink-PS Converter18/1
  Gain5/1 -> Simulink-PS Converter19/1
  Sense tL1/1(T) -> Out Bus Element/1
  Sense tR1/1(T) -> Out Bus Element5/1
  PS-Simulink Converter/1 -> Out Bus Element12/1
  PS-Simulink Converter1/1 -> Out Bus Element13/1
  PS-Simulink Converter2/1 -> Out Bus Element14/1
  PS-Simulink Converter3/1 -> Out Bus Element15/1
  PS-Simulink Converter4/1 -> Out Bus Element16/1
  Sense tL2/1(T) -> Out Bus Element1/1
  Sense tR2/1(T) -> Out Bus Element8/1
  Sense tL3/1(T) -> Out Bus Element4/1
  Sense tR3/1(T) -> Out Bus Element10/1
  PS-Simulink Converter5/1 -> Out Bus Element17/1
  connections:
  Simscape Bus1/LConn3 -- Connection Label28/LConn1
  Motor R2/RConn3 -- Motor L2/RConn3 -- C/RConn1 -- Motor R1/RConn3 -- Motor L1/RConn3 -- Motor R3/RConn3 -- Motor L3/RConn3
  Simscape Bus1/LConn4 -- Connection Label15/LConn1
  Simulink-PS Converter2/RConn1 -- Motor L1/LConn2
  Connection Label31/LConn1 -- Motor L2/RConn1
  Simscape Bus1/LConn1 -- Connection Label23/LConn1
  Sensor iL1/RConn1 -- Motor L1/LConn1
  Connection Label41/LConn1 -- Motor R3/RConn1
  Connection Label1/LConn1 -- +/RConn1 -- Sensor iL1/LConn1
  Simulink-PS Converter18/RConn1 -- Motor L3/LConn2
  Motor R2/RConn2 -- PS-Simulink Converter4/LConn1
  Simulink-PS Converter15/RConn1 -- Motor R2/LConn2
  -/RConn1 -- Connection Label3/LConn1 -- Motor L1/RConn1
  Sensor iR1/RConn1 -- Motor R1/LConn1
  Simulink-PS Converter4/RConn1 -- Motor R1/LConn2
  Connection Label8/LConn1 -- Sensor iR1/LConn1
  PS-Simulink Converter1/LConn1 -- Motor L2/RConn2
  Connection Label32/LConn1 -- Sensor iR2/LConn1
  Simscape Bus1/LConn6 -- Connection Label20/LConn1
  Connection Label33/LConn1 -- Motor R2/RConn1
  Sensor iR3/RConn1 -- Motor R3/LConn1
  PS-Simulink Converter3/LConn1 -- Motor R1/RConn2
  Motor L1/RConn2 -- PS-Simulink Converter/LConn1
  Connection Label22/LConn1 -- Gear L1/RConn1
  Simscape Bus1/LConn5 -- Connection Label16/LConn1
  Connection Label24/LConn1 -- Gear L2/RConn1
  Simulink-PS Converter14/RConn1 -- Motor L2/LConn2
  Connection Label39/LConn1 -- Motor L3/RConn1
  PS-Simulink Converter5/LConn1 -- Motor R3/RConn2
  Simulink-PS Converter19/RConn1 -- Motor R3/LConn2
  Connection Label19/LConn1 -- Gear R3/RConn1
  Sensor iR2/RConn1 -- Motor R2/LConn1
  Connection Label30/LConn1 -- Sensor iL2/LConn1
  Connection Label40/LConn1 -- Sensor iR3/LConn1
  Sensor iL3/RConn1 -- Motor L3/LConn1
  Connection Label9/LConn1 -- Motor R1/RConn1
  Sensor iL2/RConn1 -- Motor L2/LConn1
  Simscape Bus1/LConn2 -- Connection Label25/LConn1
  PS-Simulink Converter2/LConn1 -- Motor L3/RConn2
  Connection Label38/LConn1 -- Sensor iL3/LConn1
  Simscape Bus1/RConn1 -- S/RConn1
  Connection Label13/LConn1 -- Gear R1/RConn1
  Connection Label14/LConn1 -- Gear R2/RConn1
  Gear L3/RConn1 -- Connection Label21/LConn1
  Gear L1/LConn1 -- Sense tL1/LConn1
  Sense tL1/RConn1 -- Motor L1/LConn3
  Motor R1/LConn3 -- Sense tR1/RConn1
  Sense tR1/LConn1 -- Gear R1/LConn1
  Sense tL2/RConn1 -- Motor L2/LConn3
  Gear L2/LConn1 -- Sense tL2/LConn1
  Gear R2/LConn1 -- Sense tR2/LConn1
  Motor R2/LConn3 -- Sense tR2/RConn1
  Motor L3/LConn3 -- Sense tL3/RConn1
  Gear L3/LConn1 -- Sense tL3/LConn1
  Motor R3/LConn3 -- Sense tR3/RConn1
  Sense tR3/LConn1 -- Gear R3/LConn1

== system mars_rover_terrain/Rover/Chassis/Powertrain/Electrical/Power ==
  Ambient Temperature : fl_lib/Thermal/Thermal Sources/Temperature Source  temperature=273+25 K
  Battery : batteryecm_lib/Battery  Vnom=14 V  prm_dir=1  R1_dis=2 Ohm  R1_ch=2 Ohm  R1=2e-3 Ohm  prm_AH=2  AH=100 A*hr  V1=11.5 V  AH1=100/2 A*hr  prm_R2=1  R2=2000 Ohm  Tmeas=298.15 K  charge_measurement_port=simscape.enum.battery.enable.yes  prm_dyn=1  Rp1=0.005 Ohm  tau1=30 s  Rp2=0.005 Ohm  tau2=30 s  Rp3=0.005 Ohm  tau3=30 s  Rp4=0.005 Ohm  tau4=30 s  Rp5=0.005 Ohm  tau5=30 s  prm_fade=1  N_fade=100  AH_fade=45 A*hr  R1_fade=2.02 Ohm  R1_ch_fade=2.02 Ohm  V1_fade=10.35 V  prm_age=1  prm_age_OCV=1  OCV_age=0.9  SOC_age=60  Tmeas_age=298.15 K  delta_time_age_vec=[0] d  temperature_age_vec=[273] K  OCV_scaling_age=2.2134e6  OCV_offset_age=1.632e6  temp_exp_age=0.515833569 V  t_exp_age=0.75  Vnom_T2=12 V  R1_T2=2e-2 Ohm  R1_T2_dis=2.2 Ohm  R1_T2_ch=2.2 Ohm  V1_T2=11.4 V  R2_T2=2200 Ohm  Rp1_T2=0.005 Ohm  tau1_T2=30 s  Rp2_T2=0.005 Ohm  tau2_T2=30 s  Rp3_T2=0.005 Ohm  tau3_T2=30 s  Rp4_T2=0.005 Ohm  tau4_T2=30 s  Rp5_T2=0.005 Ohm  tau5_T2=30 s  Tmeas2=273.15 K  thermal_port=simscape.enum.thermaleffects.model  thermal_mass=30000 J/K  i_specify=off  i_priority=None  i=0 A  i_nominal_specify=off  i_nominal_value=1  i_nominal_unit=A  v_specify=off  v_priority=None  v=0 V  v_nominal_specify=off  v_nominal_value=1  v_nominal_unit=V  charge_specify=on  charge_priority=High  charge=100 A*hr  charge_nominal_specify=off  charge_nominal_value=1  charge_nominal_unit=A*hr  num_cycles_specify=off  num_cycles_priority=High  num_cycles=0  num_cycles_nominal_specify=off  num_cycles_nominal_value=1  num_cycles_nominal_unit=1  temperature_specify=on  temperature_priority=High  temperature=288.15 K  temperature_nominal_specify=off  temperature_nominal_value=1  temperature_nominal_unit=K
      settings: LogSimulationData=on  InternalSimscapePortConfiguration="{\"Bottom\":[],\"Left\":[{\"id\":\"p\",\"label\":\"+\",\"type\":\"foundation.electrical.electrical\"},{\"id\":\"q\",\"label\":\"q\",\"type\":\"output\"}],\"Right\":[{\"id\":\"n\",\"label\":\"-\",\"type\":\"foundation.electrical.electrical\"},{\"id\":\"H\",\"label\":\"H\",\"type\":\"foundation.thermal.thermal\"}],\"Top\":[]}"
  Convective Heat Transfer : fl_lib/Thermal/Thermal Elements/Convective Heat Transfer  thermal_type=foundation.enum.constant_variable.constant  area=1e-4 m^2  heat_tr_coeff=20 W/(m^2 * K)  min_heat_tr_coeff=1e-3 W/(K*m^2)  T_specify=off  T_priority=None  T=0 K  T_nominal_specify=off  T_nominal_value=1  T_nominal_unit=K  Q_specify=off  Q_priority=None  Q=0 W  Q_nominal_specify=off  Q_nominal_value=1  Q_nominal_unit=W
  Electrical Reference : fl_lib/Electrical/Electrical Elements/Electrical Reference
  PS-Simulink Converter : nesl_utility/PS-Simulink Converter  PhysicalDomain=network_engine_domain  SubClassName=ps_output  LeftPortType=input  RightPortType=output  PseudoPeriodic=off  Frequencies=[]  VectorFormat=1-D array  Unit=hr*A  AffineConversion=off
  Sensing Temperature : Subsystem
  + : PMIOPort  Side=Right
  - : PMIOPort  Port=2  Side=Right
  Out Bus Element4 : Outport  PortName=m  Element=SOC
  Out Bus Element5 : Outport  PortName=m  Element=degC
  wires:
  Sensing Temperature/1(T) -> Out Bus Element5/1
  PS-Simulink Converter/1 -> Out Bus Element4/1
  connections:
  Battery/RConn1 -- Electrical Reference/LConn1 -- -/RConn1
  Battery/LConn1 -- +/RConn1
  Convective Heat Transfer/RConn1 -- Ambient Temperature/LConn1
  Battery/RConn2 -- Convective Heat Transfer/LConn1 -- Sensing Temperature/LConn1
  PS-Simulink Converter/LConn1 -- Battery/LConn2
